simulink model "EV_Truck_Model"  (R2022b)
settings: Solver=FixedStepAuto  StartTime=0  StopTime=26553  FixedStep=0.1  RelTol=1e-3
model workspace (MAT data in the model file):
  ADAS_MaxAccel = 2
  ADAS_MaxDecel = 2.5
  Adas_on_off = 0
  Batt_cap_ah : Simulink.Parameter (value not decoded)
  Batt_rist_r0 : Simulink.Parameter (value not decoded)
  Batt_soc_s0 : Simulink.Parameter (value not decoded)
  Batt_volt_v0 : Simulink.Parameter (value not decoded)
  Motor_eff_100 : Simulink.Parameter (value not decoded)
  Motor_eff_190 : Simulink.Parameter (value not decoded)
  Motor_eff_95 : Simulink.Parameter (value not decoded)
  Motor_rpm_100 : Simulink.Parameter (value not decoded)
  Motor_rpm_190 : Simulink.Parameter (value not decoded)
  Motor_rpm_95 : Simulink.Parameter (value not decoded)
  Motor_torque_pos_100 : Simulink.Parameter (value not decoded)
  Motor_torque_pos_190 : Simulink.Parameter (value not decoded)
  Motor_torque_pos_95 : Simulink.Parameter (value not decoded)
  Motor_trq_190 : Simulink.Parameter (value not decoded)
  Motor_trq_95 : Simulink.Parameter (value not decoded)
  Sim_step = 0.1
  Test_DriveCycle = 0
  Trans_ratio = 6.142
  Veh_cog_fx = 1.69543
  Veh_cog_h = 0.605887
  Veh_cog_rx = 2.11956
  Veh_diff = 6.7
  Veh_whl_crr = 0.01
  Veh_whl_k = 180000
  Veh_whl_radius = 0.35
symbols that are objects in the model workspace (value not decoded): Motor_eff_100, Motor_eff_190, Motor_eff_95, Motor_rpm_100, Motor_rpm_190, Motor_rpm_95, Motor_torque_pos_100, Motor_torque_pos_190, Motor_torque_pos_95, Motor_trq_190, Motor_trq_95
undefined symbols (not defined in the file): Batt_soc_init, canChannel, Elec_aux_sw, Elec_rgn_sw, Power_option, speed, time, Veh_mass
libraries: batteryecm_lib x170, simulink x14, canmsglib x9, canlib x7, autolibshared x5, nesl_utility x4, fl_lib x3, drivingvehiclecontroller x3, hdlsllib x3, sim3dlib x1, sim3dautolib x1, vrlib x1
(part 4 of 11)

== system EV_Truck_Model/Vehicle Dynamics System/Power Delivery and Braking System/GearBox ==
  AxleTorque : Inport
  Chart : Stateflow chart  Commented=on  TreatAsAtomicUnit=on
  DrivingTorque : Outport
  wires:
  AxleTorque/1 -> DrivingTorque/1
